simulink model "lab6"  (R2025b)
settings: Solver=VariableStepAuto  StartTime=0.0  StopTime=100  RelTol=1e-3
undefined symbols (not defined in the file): gamma, k_0, k_1
settings Model: Creator=Nickolay  LastModifiedBy=Nickolay

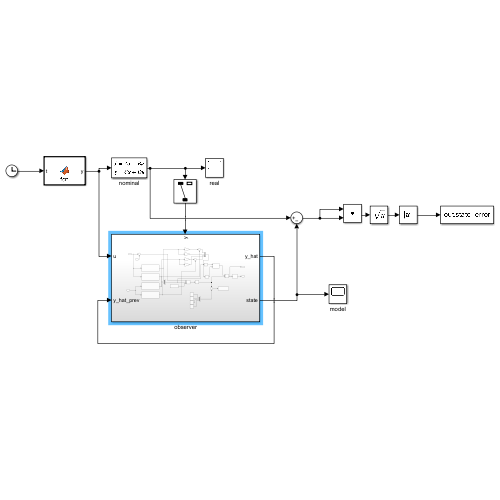
[thumbnail: Simulink's stored preview of the top-level diagram]
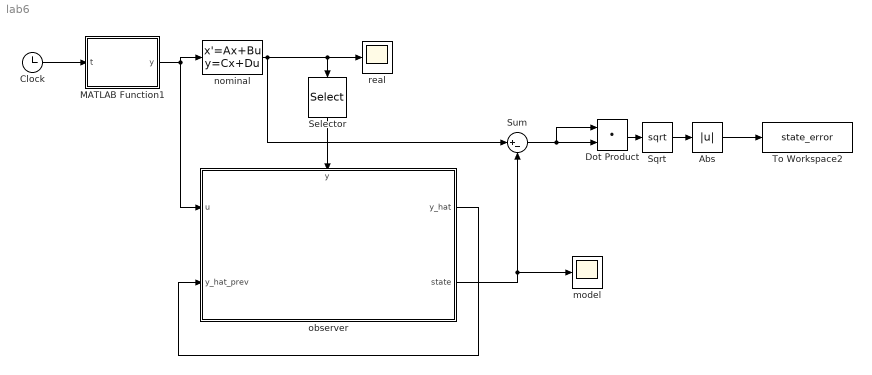
== system lab6 ==
  Abs : Abs  SaturateOnIntegerOverflow=off
  Clock : Clock
  Dot Product : DotProduct  OutDataTypeStr=Inherit: Inherit via internal rule
  MATLAB Function1 : MATLAB Function  TreatAsAtomicUnit=on
  Selector : Selector  InputPortWidth=2  IndexOptions=Index vector (dialog)  Indices=1  OutputSizes=1
  Sqrt : Sqrt
  Sum : Sum  Inputs=|+-
  To Workspace2 : ToWorkspace  VariableName=state_error  SaveFormat=Timeseries  SampleTime=-1
  model : Scope
      settings: ActiveDisplayYMinimum=-33.141911664691982  ActiveDisplayYMaximum=30.748024729439155
  nominal : StateSpace  A=[-1 1; -1 0]  B=[1; 2]  C=eye(2)  D=zeros(2, 1)  InitialCondition=0
  observer : Subsystem
      settings: PortSchema="{\"entries\":[{\"content\":{\"sides\":[{\"content\":{\"connectorIds\":[\"In1\",\"In2\"]},\"type\":\"ConnectorPlacement.EquallySpacedRectSide\",\"uuid\":\"e7575c5d-fbef-47fc-b52b-9edd90a7515c\"},{\"content\":{\"connectorIds\":[\"Out1\",\"Out2\"],\"side\":\"RIGHT\"},\"type\":\"ConnectorPlacement.EquallySpacedRectSide\",\"uuid\":\"d1208134-eb77-47e1-bcad-d07747fe6552\"},{\"content\":{\"connectorIds\":[\"In3\"],\"side\":\"TOP\"},\"type\":\"ConnectorPlacement.EquallySpacedRectSide\",\"uuid\":\"74b80bf8-5acc-4343-b9c8-665d308db7dc\"}]},\"type\":\"ConnectorPlacement.EquallySpacedConnector\",\"uuid\":\"0f2872db-0ef9-49b2-bee1-7b09b6b4b057\"}],\"packageUris\":[\"http://schema.mathworks.com/mf0/Connector/R2020b\"],\"version\":\"1.0\"}"
  real : Scope
      settings: ActiveDisplayYMinimum=-33.463635422591828  ActiveDisplayYMaximum=26.129453060204327
  wires:
  Clock/1 -> MATLAB Function1/1(t)
  observer/1(y_hat) -> observer/2(y_hat_prev)
  Selector/1 -> observer/3(y)
  MATLAB Function1/1(y) -> nominal/1, observer/1(u)
  observer/2(state) -> model/1, Sum/2
  Sum/1 -> Dot Product/1, Dot Product/2
  nominal/1 -> Sum/1, real/1, Selector/1
  Abs/1 -> To Workspace2/1
  Dot Product/1 -> Sqrt/1
  Sqrt/1 -> Abs/1

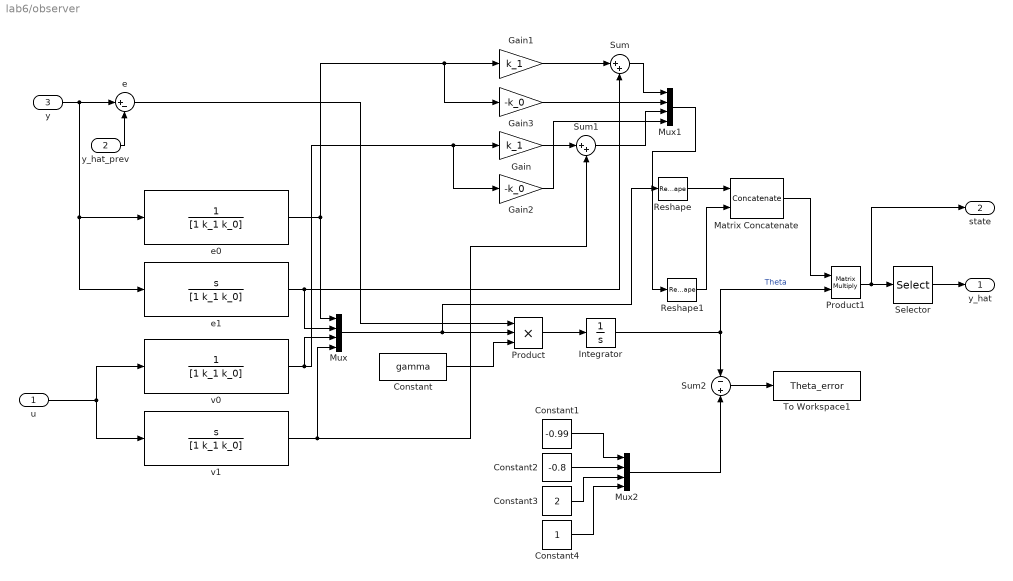
== system lab6/observer ==
  u : Inport
  y_hat_prev : Inport  Port=2
  y : Inport  Port=3
  Constant : Constant  Value=gamma
  Constant1 : Constant  Value=-0.99
  Constant2 : Constant  Value=-0.8
  Constant3 : Constant  Value=2
  Constant4 : Constant
  Gain : Gain  Gain=k_1
  Gain1 : Gain  Gain=k_1
  Gain2 : Gain  Gain=-k_0
  Gain3 : Gain  Gain=-k_0
  Integrator : Integrator
  Matrix Concatenate : Concatenate  Mode=Multidimensional array
  Mux : Mux
  Mux1 : Mux
  Mux2 : Mux
  Product : Product  Inputs=3
  Product1 : Product  Multiplication=Matrix(*)
  Reshape : Reshape  OutputDimensionality=Row vector (2-D)
  Reshape1 : Reshape  OutputDimensionality=Row vector (2-D)
  Selector : Selector  InputPortWidth=2  IndexOptions=Index vector (dialog)  Indices=1  OutputSizes=1
  Sum : Sum  Inputs=|++
  Sum1 : Sum  Inputs=|++
  Sum2 : Sum  Inputs=-+
  To Workspace1 : ToWorkspace  VariableName=Theta_error  SaveFormat=Timeseries  SampleTime=-1
  e : Sum  Inputs=|+-
  e0 : TransferFcn  Denominator=[1 k_1 k_0]
  e1 : TransferFcn  Numerator=[1 0]  Denominator=[1 k_1 k_0]
  v0 : TransferFcn  Denominator=[1 k_1 k_0]
  v1 : TransferFcn  Numerator=[1 0]  Denominator=[1 k_1 k_0]
  y_hat : Outport
  state : Outport  Port=2
  wires:
  y/1 -> e1/1, e0/1, e/1
  y_hat_prev/1 -> e/2
  u/1 -> v0/1, v1/1
  e0/1 -> Gain3/1, Gain1/1, Mux/1
  e1/1 -> Sum/2, Mux/2
  v0/1 -> Gain2/1, Gain/1, Mux/3
  v1/1 -> Sum1/2, Mux/4
  e/1 -> Product/1
  Mux/1 -> Reshape/1, Product/2
  Constant/1 -> Product/3
  Product/1 -> Integrator/1
  Integrator/1 -> Product1/2, Sum2/1  "Theta"
  Gain1/1 -> Sum/1
  Sum/1 -> Mux1/1
  Gain3/1 -> Mux1/2
  Gain/1 -> Sum1/1
  Sum1/1 -> Mux1/3
  Gain2/1 -> Mux1/4
  Mux1/1 -> Reshape1/1
  Reshape1/1 -> Matrix Concatenate/2
  Reshape/1 -> Matrix Concatenate/1
  Matrix Concatenate/1 -> Product1/1
  Sum2/1 -> To Workspace1/1
  Constant1/1 -> Mux2/1
  Constant2/1 -> Mux2/2
  Constant4/1 -> Mux2/4
  Constant3/1 -> Mux2/3
  Mux2/1 -> Sum2/2
  Selector/1 -> y_hat/1
  Product1/1 -> state/1, Selector/1

== matlab function lab6/MATLAB Function1 ==
  data: t input; y output; task1 parameter
function y = fcn(t, task1)

y = 10*sin(t);

if task1 ~= 1
    y = y + 5*cos(2*t) + 4*cos(4*t) + 3*cos(8*t);
end

end
